simulink model "PerceptionAndGuidance"  (R2026b)
settings: Solver=ode3  StopTime=TFinal
PreLoadFcn:
  | InitVars;
libraries: raspberrypiutilitieslib x2, raspberrypiCommlib x2, simulink x1
settings Model: Creator=The MathWorks, Inc.  LastModifiedBy=rbhan
settings SolverCC: AutoInsertRateTranBlk=on  PositivePriorityOrder=on
settings OptimizationCC: DifferentSizesBufferReuse=on  EfficientTunableParamExpr=on  EnhancedBackFolding=on  MaxStackSize=200000  OptimizationCustomize=off  OptimizeBlockOrder=speed  PassReuseOutputArgsAs=Individual arguments  RemoveInternalMemoryZeroInit=on  RemoveRootLevelIOMemoryZeroInit=on
settings DebuggingCC: ParameterPrecisionLossMsg=none  ParameterTunabilityLossMsg=error
settings HardwareCC: ProdHWDeviceType=ARM Compatible->ARM Cortex-A (32-bit)  ProdLargestAtomicFloat=Double  ProdLargestAtomicInteger=Long  ProdLongLongMode=on
settings ModelReferenceCC: PropagateVarSize=During execution
settings RTWCC: BuildConfiguration=Faster Runs  Description=Embedded Coder  SystemTargetFile=ert.tlc  TemplateMakefile=ert_default_tmf
settings CodeAppCC: ForceParamTrailComments=on  IgnoreCustomStorageClasses=off  InsertBlockDesc=on  OperatorAnnotations=on  SFDataObjDesc=on  SimulinkDataObjDesc=on
settings ERTTargetCC: CodeReplacementLibrary=ARM Cortex-A CMSIS  ExtModeIntrfLevel=Level2 - Open  ExtModeMexFile=ext_xcp  ExtModeStaticAlloc=on  SupportVariableSizeSignals=on

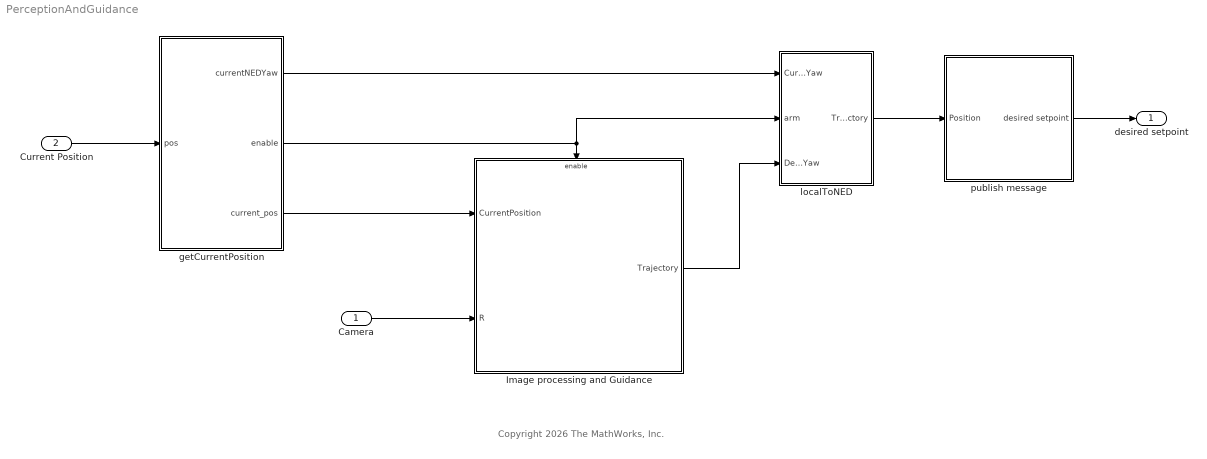
== system PerceptionAndGuidance ==
  note: Copyright 2026 The MathWorks, Inc.
  Camera : Inport  OutDataTypeStr=uint8  PortDimensions=[120 160 3]
  Current Position : Inport  Port=2  OutDataTypeStr=double  PortDimensions=4
  Image processing and Guidance : Subsystem
  getCurrentPosition : Subsystem  Variant=on
  localToNED : Subsystem
  publish message : Subsystem  Variant=on
  desired setpoint : Outport  OutDataTypeStr=Bus: desiredTargetSetpoints
  wires:
  localToNED/1(Trajectory) -> publish message/1(Position)
  getCurrentPosition/1(currentNEDYaw) -> localToNED/1(CurrentNEDYaw)
  Image processing and Guidance/1(Trajectory) -> localToNED/3(DesiredPosAndYaw)
  getCurrentPosition/2(enable) -> Image processing and Guidance/Enable, localToNED/2(arm)
  Camera/1 -> Image processing and Guidance/2(R)
  Current Position/1 -> getCurrentPosition/1(pos)
  getCurrentPosition/3(current_pos) -> Image processing and Guidance/1(CurrentPosition)
  publish message/1(desired setpoint) -> desired setpoint/1

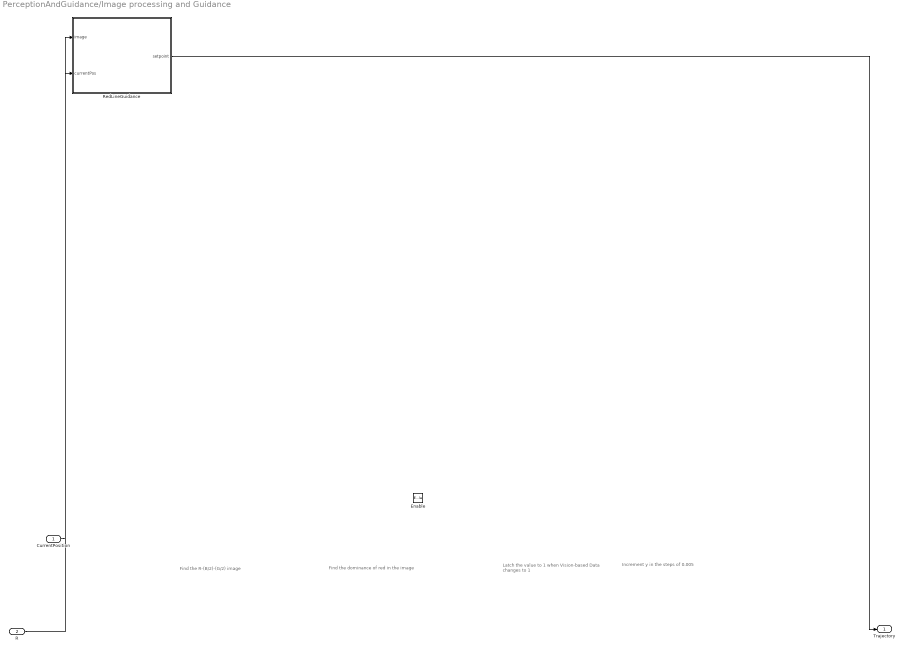
== system PerceptionAndGuidance/Image processing and Guidance ==
  note: Find the dominance of red in the image
  note: Increment y in the steps of 0.005
  note: Find the R-(B/2)-(G/2) image
  note: Latch the value to 1 when
      | Vision-based Data changes to 1
  CurrentPosition : Inport  OutDataTypeStr=double  PortDimensions=4
  R : Inport  Port=2  OutDataTypeStr=uint8  PortDimensions=[120 160 3]
  Enable : EnablePort
  RedLineGuidance : MATLAB Function  TreatAsAtomicUnit=on
  Trajectory : Outport
  wires:
  R/1 -> RedLineGuidance/1(image)
  CurrentPosition/1 -> RedLineGuidance/2(currentPos)
  RedLineGuidance/1(setpoint) -> Trajectory/1

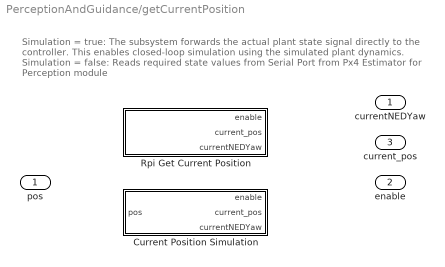
== system PerceptionAndGuidance/getCurrentPosition ==
  note: Simulation = true:
      | The subsystem forwards the actual plant state signal directly to the controller. This enables closed-loop simulation using the simulated plant dynamics.
      |
      | Simulation = false:
      | Reads required state values from Serial Port from Px4 Estimator for Perception module
  pos : Inport  PortDimensions=[1 4]
  Current Position Simulation : Subsystem  VariantControl=Simulation == true
  Rpi Get Current Position : Subsystem  VariantControl=Simulation == false
  currentNEDYaw : Outport
  enable : Outport  Port=2
  current_pos : Outport  Port=3

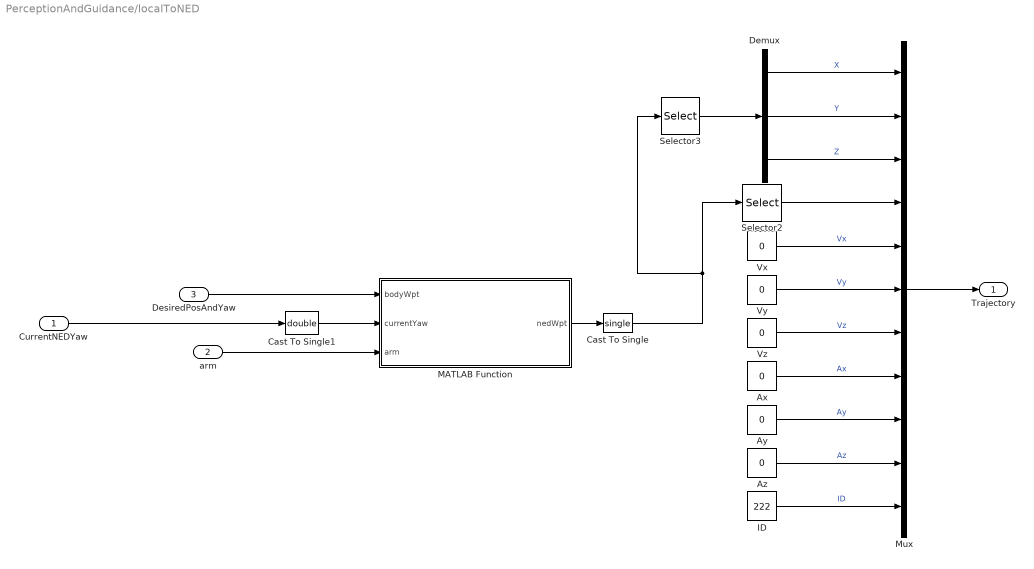
== system PerceptionAndGuidance/localToNED ==
  CurrentNEDYaw : Inport
  arm : Inport  Port=2
  DesiredPosAndYaw : Inport  Port=3
  Ax : Constant  Value=0  OutDataTypeStr=single  SampleTime=-1
  Ay : Constant  Value=0  OutDataTypeStr=single  SampleTime=-1
  Az : Constant  Value=0  OutDataTypeStr=single  SampleTime=-1
  Cast To Single : DataTypeConversion  OutDataTypeStr=single  SaturateOnIntegerOverflow=off  RndMeth=Floor
  Cast To Single1 : DataTypeConversion  OutDataTypeStr=double  SaturateOnIntegerOverflow=off  RndMeth=Floor
  Demux : Demux  Outputs=3
  ID : Constant  Value=222  OutDataTypeStr=single  SampleTime=-1
  MATLAB Function : MATLAB Function  TreatAsAtomicUnit=on
  Mux : Mux  Inputs=11
  Selector2 : Selector  InputPortWidth=4  IndexOptions=Index vector (dialog)  Indices=4  OutputSizes=1
  Selector3 : Selector  InputPortWidth=4  IndexOptions=Index vector (dialog)  Indices=[1:3]  OutputSizes=1
  Vx : Constant  Value=0  OutDataTypeStr=single  SampleTime=-1
  Vy : Constant  Value=0  OutDataTypeStr=single  SampleTime=-1
  Vz : Constant  Value=0  OutDataTypeStr=single  SampleTime=-1
  Trajectory : Outport
  wires:
  Selector3/1 -> Demux/1
  Mux/1 -> Trajectory/1
  Demux/2 -> Mux/2  "Y"
  Demux/3 -> Mux/3  "Z"
  Selector2/1 -> Mux/4
  Cast To Single/1 -> Selector3/1, Selector2/1
  ID/1 -> Mux/11  "ID"
  Demux/1 -> Mux/1  "X"
  Vx/1 -> Mux/5  "Vx"
  Vy/1 -> Mux/6  "Vy"
  Az/1 -> Mux/10  "Az"
  Vz/1 -> Mux/7  "Vz"
  Ay/1 -> Mux/9  "Ay"
  MATLAB Function/1(nedWpt) -> Cast To Single/1
  Ax/1 -> Mux/8  "Ax"
  DesiredPosAndYaw/1 -> MATLAB Function/1(bodyWpt)
  CurrentNEDYaw/1 -> Cast To Single1/1
  Cast To Single1/1 -> MATLAB Function/2(currentYaw)
  arm/1 -> MATLAB Function/3(arm)

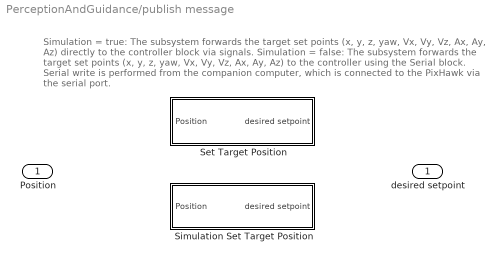
== system PerceptionAndGuidance/publish message ==
  note: Simulation = true:
      | The subsystem forwards the target set points (x, y, z, yaw, Vx, Vy, Vz, Ax, Ay, Az) directly to the controller block via signals.
      |
      | Simulation = false:
      | The subsystem forwards the target set points (x, y, z, yaw, Vx, Vy, Vz, Ax, Ay, Az) to the controller using the Serial block. Serial write is performed from the companion computer, which is connected to the PixHawk via the serial port.
  Position : Inport
  Set Target Position : Subsystem  VariantControl=Simulation == false
  Simulation Set Target Position : Subsystem  VariantControl=Simulation == true
  desired setpoint : Outport

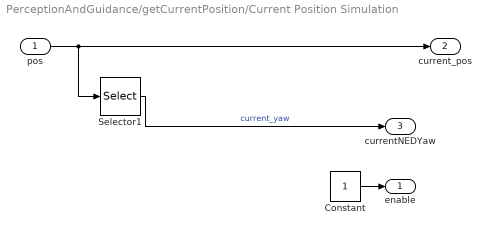
== system PerceptionAndGuidance/getCurrentPosition/Current Position Simulation ==
  pos : Inport
  Constant : Constant  SampleTime=-1
  Selector1 : Selector  InputPortWidth=4  IndexOptions=Index vector (dialog)  Indices=4  OutputSizes=1
  enable : Outport
  current_pos : Outport  Port=2
  currentNEDYaw : Outport  Port=3
  wires:
  pos/1 -> current_pos/1, Selector1/1
  Constant/1 -> enable/1
  Selector1/1 -> currentNEDYaw/1  "current_yaw"

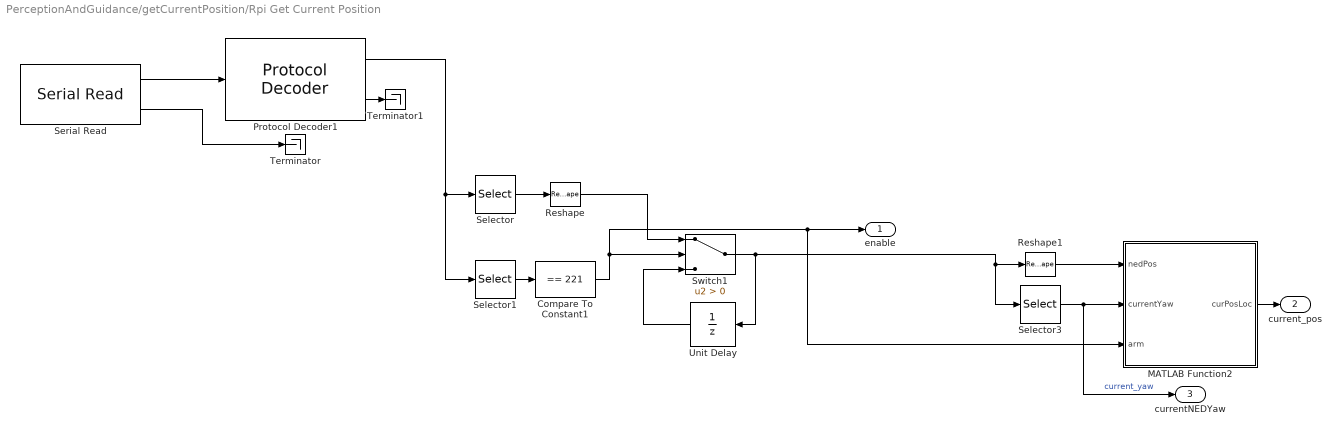
== system PerceptionAndGuidance/getCurrentPosition/Rpi Get Current Position ==
  Compare To Constant1 : simulink/Logic and Bit Operations/Compare To Constant  relop===  const=221  OutDataTypeStr=boolean
  MATLAB Function2 : MATLAB Function  TreatAsAtomicUnit=on
  Protocol Decoder1 : raspberrypiutilitieslib/Protocol Decoder  IsParseCSV=off  Header=[123]  FieldTable={ 'Field1', '5', 'single', 'Little endian' }  IsVariableSizeLastField=off  MaxVariableSizeFieldLength=[]  IsChecksumRequired=off  ChecksumAlgorithm=XOR of bytes  ChecksumSize=[]  TerminatorOption=<none>  CustomTerminatorVal=[]  IsInputLengthAvailable=off
  Reshape : Reshape
  Reshape1 : Reshape  OutputDimensionality=Customize  OutputDimensions=[4,1]
  Selector : Selector  InputPortWidth=5  IndexOptions=Index vector (dialog)  Indices=[1:4]  OutputSizes=1
  Selector1 : Selector  InputPortWidth=5  IndexOptions=Index vector (dialog)  Indices=[5]  OutputSizes=1
  Selector3 : Selector  InputPortWidth=4  IndexOptions=Index vector (dialog)  Indices=4  OutputSizes=1
  Serial Read : raspberrypiCommlib/Serial Read  board=Pi Zero W  SCIModule_=/dev/ttyACM0  Baudrate_=115200  Parity=None  StopBits_=1  HardwareFlowControl=None  ByteOrder=LittleEndian  DataLength=21  DataType=uint8  OutputStatus=on  SampleTime=0.1  blockPlatform=RaspberryPi
  Switch1 : Switch  Criteria=u2 > Threshold  SaturateOnIntegerOverflow=off  InputSameDT=off
  Terminator : Terminator
  Terminator1 : Terminator
  Unit Delay : UnitDelay  InitialCondition=[0 0 0 0]'  SampleTime=-1
  enable : Outport
  current_pos : Outport  Port=2
  currentNEDYaw : Outport  Port=3
  wires:
  Unit Delay/1 -> Switch1/3
  Serial Read/1 -> Protocol Decoder1/1
  Serial Read/2 -> Terminator/1
  Protocol Decoder1/1 -> Selector1/1, Selector/1
  Selector1/1 -> Compare To Constant1/1
  Selector/1 -> Reshape/1
  Reshape/1 -> Switch1/1
  Protocol Decoder1/2 -> Terminator1/1
  Selector3/1 -> currentNEDYaw/1, MATLAB Function2/2(currentYaw)  "current_yaw"
  Compare To Constant1/1 -> MATLAB Function2/3(arm), enable/1, Switch1/2
  Switch1/1 -> Unit Delay/1, Selector3/1, Reshape1/1
  Reshape1/1 -> MATLAB Function2/1(nedPos)
  MATLAB Function2/1(curPosLoc) -> current_pos/1

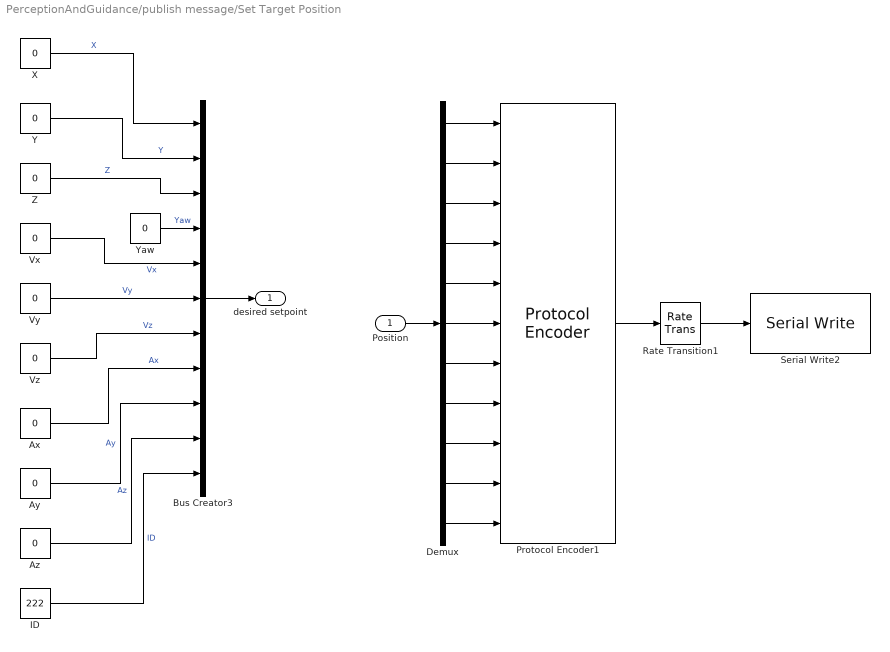
== system PerceptionAndGuidance/publish message/Set Target Position ==
  Position : Inport
  Ax : Constant  Value=0  SampleTime=-1
  Ay : Constant  Value=0  SampleTime=-1
  Az : Constant  Value=0  SampleTime=-1
  Bus Creator3 : BusCreator  Inputs=11  OutDataTypeStr=Bus: desiredTargetSetpoints
  Demux : Demux  Outputs=11
  ID : Constant  Value=222  SampleTime=-1
  Protocol Encoder1 : raspberrypiutilitieslib/Protocol Encoder  Header=[134]  FieldTable={ 'Field1', '1', 'single', 'Little endian'; 'Field2', '1', 'single', 'Little endian'; 'Field3', '1', 'single', 'Little endian'; 'Field4', '1', 'single', 'Little endian'; 'Field5', '1', 'single', 'Little endian'; 'Field6', '1', 'single', 'Little endian'; 'Field7', '1', 'single', 'Little endian'; 'Field8', '1', 'single', 'Little endian'; 'Field9', '1', 'single', 'Little endian'; 'Field10', '1', 'single', 'Little endian'; 'Field11', '1', 'single', 'Little endian' }  IsChecksumRequired=off  ChecksumAlgorithm=XOR of bytes  ChecksumSize=[]  TerminatorOption=<none>  CustomTerminatorVal=[]
  Rate Transition1 : RateTransition  OutPortSampleTime=1/10
  Serial Write2 : raspberrypiCommlib/Serial Write  board=Pi Zero W  SCIModule_=/dev/ttyACM0  Baudrate_=115200  Parity=None  StopBits_=1  HardwareFlowControl=None  ByteOrder=LittleEndian  OutputStatus=off  blockPlatform=RaspberryPi
  Vx : Constant  Value=0  SampleTime=-1
  Vy : Constant  Value=0  SampleTime=-1
  Vz : Constant  Value=0  SampleTime=-1
  X : Constant  Value=0  SampleTime=-1
  Y : Constant  Value=0  SampleTime=-1
  Yaw : Constant  Value=0  SampleTime=-1
  Z : Constant  Value=0  SampleTime=-1
  desired setpoint : Outport  OutDataTypeStr=Bus: desiredTargetSetpoints
  wires:
  Ax/1 -> Bus Creator3/8  "Ax"
  X/1 -> Bus Creator3/1  "X"
  Y/1 -> Bus Creator3/2  "Y"
  Z/1 -> Bus Creator3/3  "Z"
  Ay/1 -> Bus Creator3/9  "Ay"
  Vx/1 -> Bus Creator3/5  "Vx"
  Vy/1 -> Bus Creator3/6  "Vy"
  Vz/1 -> Bus Creator3/7  "Vz"
  Az/1 -> Bus Creator3/10  "Az"
  ID/1 -> Bus Creator3/11  "ID"
  Bus Creator3/1 -> desired setpoint/1
  Rate Transition1/1 -> Serial Write2/1
  Protocol Encoder1/1 -> Rate Transition1/1
  Demux/1 -> Protocol Encoder1/1
  Demux/2 -> Protocol Encoder1/2
  Demux/3 -> Protocol Encoder1/3
  Demux/4 -> Protocol Encoder1/4
  Demux/5 -> Protocol Encoder1/5
  Demux/6 -> Protocol Encoder1/6
  Demux/7 -> Protocol Encoder1/7
  Demux/8 -> Protocol Encoder1/8
  Demux/9 -> Protocol Encoder1/9
  Demux/10 -> Protocol Encoder1/10
  Demux/11 -> Protocol Encoder1/11
  Position/1 -> Demux/1
  Yaw/1 -> Bus Creator3/4  "Yaw"

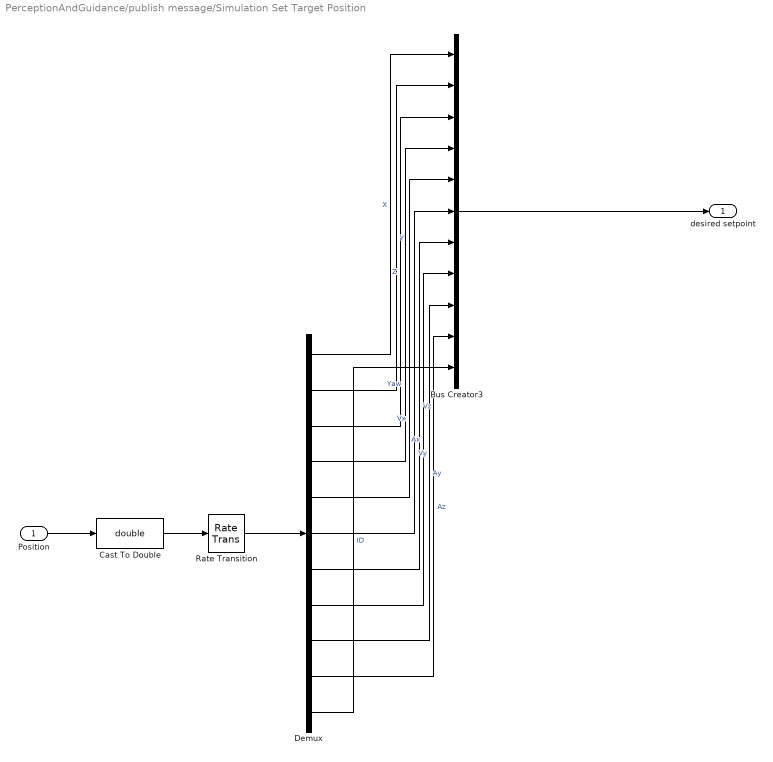
== system PerceptionAndGuidance/publish message/Simulation Set Target Position ==
  Position : Inport
  Bus Creator3 : BusCreator  Inputs=11  OutDataTypeStr=Bus: desiredTargetSetpoints
  Cast To Double : DataTypeConversion  OutDataTypeStr=double  SaturateOnIntegerOverflow=off  RndMeth=Floor
  Demux : Demux  Outputs=11
  Rate Transition : RateTransition  OutPortSampleTime=0.2
  desired setpoint : Outport  OutDataTypeStr=Bus: desiredTargetSetpoints
  wires:
  Demux/1 -> Bus Creator3/1  "X"
  Demux/2 -> Bus Creator3/2  "Y"
  Demux/3 -> Bus Creator3/3  "Z"
  Demux/4 -> Bus Creator3/4  "Yaw"
  Demux/5 -> Bus Creator3/5  "Vx"
  Demux/6 -> Bus Creator3/6  "Vy"
  Demux/7 -> Bus Creator3/7  "Vz"
  Demux/8 -> Bus Creator3/8  "Ax"
  Demux/9 -> Bus Creator3/9  "Ay"
  Demux/10 -> Bus Creator3/10  "Az"
  Demux/11 -> Bus Creator3/11  "ID"
  Position/1 -> Cast To Double/1
  Rate Transition/1 -> Demux/1
  Cast To Double/1 -> Rate Transition/1
  Bus Creator3/1 -> desired setpoint/1

== matlab function PerceptionAndGuidance/getCurrentPosition/Rpi Get Current Position/MATLAB Function2 ==
  data: nedPos input; curPosLoc output; currentYaw input; arm input
function curPosLoc = ned2body_waypoint(nedPos, currentYaw, arm)
% nedPos: 1x4 [x_ned, y_ned, z, yaw_ned]
% currentYaw: scalar (current yaw from PX4, in radians)
% arm: boolean (true if vehicle is armed)
% Output: 1x4 [x_body, y_body, z, yaw_body]

persistent yaw0 isLatched

if isempty(yaw0)
    yaw0 = single(0);
end
if isempty(isLatched)
    isLatched = false;
end

x_n = nedPos(1);
y_n = nedPos(2);
z_n = nedPos(3);
yaw_n = nedPos(4);

if arm && ~isLatched
    yaw0 = currentYaw;    % latch yaw when arming occurs
    isLatched = true;
elseif ~arm
    isLatched = false;    % reset latch if disarmed
end

if isLatched
    % Transform to body frame relative to yaw0
    x_b =  x_n * cos(yaw0) + y_n * sin(yaw0);
    y_b = -x_n * sin(yaw0) + y_n * cos(yaw0);
    yaw_b = wrapToPi(yaw_n - yaw0);
    curPosLoc = [x_b; y_b; z_n; yaw_b];
else
    % Not armed: just forward readings (no transform)
    curPosLoc = [x_n; y_n; z_n; yaw_n];
end
end

== matlab function PerceptionAndGuidance/localToNED/MATLAB Function ==
  data: bodyWpt input; nedWpt output; currentYaw input; arm input
function nedWpt = body2ned_waypoint(bodyWpt, currentYaw, arm)
%#codegen
nedWpt = double(reshape(bodyWpt, 4, 1));
end

== matlab function PerceptionAndGuidance/Image processing and Guidance/RedLineGuidance ==
  data: image input uint8 size=[120 160 3]; setpoint output double size=4; currentPos input double size=4
function setpoint = RedLineGuidance(image, currentPos)
%#codegen
% REDLINEGUIDANCE Robust closed-loop perception and guidance for MATLAB Minidrone Red Line Follower
%
% Fully autonomous guidance system designed to follow arbitrary red line tracks regardless of
% geometry: normal corners (90 deg), sharp acute corners (45-60 deg / hairpins), obtuse turns,
% smooth curves, line gaps, and distractors, with precision alignment and landing on the destination circle.
%
% Inputs:
%   image:      120x160x3 uint8 downward camera frame
%   currentPos: [X; Y; Z; yaw] drone state in NED frame
%
% Output:
%   setpoint:   [X_cmd; Y_cmd; Z_cmd; yaw_cmd] in NED frame

persistent state x_cmd y_cmd z_cmd yaw_cmd is_init
persistent last_valid_yaw loss_timer takeoff_timer align_timer landed_timer
persistent x0 y0 yaw0 circle_x circle_y
persistent corner_x corner_y corner_turn_dir turn_start_yaw
persistent circle_confirm_timer corner_cooldown incoming_yaw
persistent turn_score

% State definitions:
% 0: TAKEOFF / CLIMB
% 1: TRACK (Lookahead pursuit for straight lines and gentle curves)
% 2: APPROACH_CORNER (Straight-line deceleration into corner vertex, zero lateral drift, zero overshoot)
% 3: CORNER_TURN (In-place yaw rotation holding corner vertex, handles 45-160 deg turns)
% 4: GAP_RECOVER (Crawl along last heading if line temporarily lost)
% 5: ALIGN_CIRCLE (Precision 2D centering over destination circle)
% 6: LAND (Active descent with closed-loop centering)
% 7: LANDED (Touchdown hold)

dt = 0.20;          % Camera frame period (5 Hz)
CRUISE_ALT = -0.80; % Cruise altitude (0.8m above ground)

if isempty(is_init)
    state = 0;
    x0 = currentPos(1);
    y0 = currentPos(2);
    yaw0 = currentPos(4);
    x_cmd = x0;
    y_cmd = y0;
    z_cmd = CRUISE_ALT;
    yaw_cmd = yaw0;
    last_valid_yaw = yaw0;
    incoming_yaw = yaw0;
    circle_x = x0;
    circle_y = y0;
    corner_x = x0;
    corner_y = y0;
    corner_turn_dir = 1;
    turn_start_yaw = yaw0;
    loss_timer = 0;
    takeoff_timer = 0;
    align_timer = 0;
    landed_timer = 0;
    circle_confirm_timer = 0;
    corner_cooldown = 0;
    turn_score = 0;
    is_init = true;
end

% Decrement corner cooldown timer
if corner_cooldown > 0
    corner_cooldown = max(0, corner_cooldown - dt);
end

% Extract RGB color channels
R = double(image(:,:,1));
G = double(image(:,:,2));
B = double(image(:,:,3));

% 1. Robust Red Pixel Segmentation
% Rejects gravel floor (grey/green), yellow distractors (R~G), blue distractors, and shadows
is_red = (R > 75) & ...
         (R - G > 25) & ...
         (R - B > 25) & ...
         (R ./ max(G + B, 1) > 0.65);

nRed = sum(is_red(:));

% Altitude-adaptive metric scaling (meters per pixel)
curr_h = max(-currentPos(3), 0.15);
scale = 0.00432 * (curr_h / 0.80);

% 2. Image Feature Extraction
% Camera frame geometry:
% Row 1 = Forward (+X body), Row 120 = Rear (-X body), Row 60 = Nadir (drone center)
% Col 1 = Left (-Y body), Col 160 = Right (+Y body), Col 80 = Centerline

[rAll, cAll] = find(is_red);
if ~isempty(rAll)
    c_all = mean(cAll);
    r_all = mean(rAll);
    min_c = min(cAll);
    max_c = max(cAll);
    min_r = min(rAll);
    max_r = max(rAll);
    r_span = max_r - min_r;
    c_span = max_c - min_c;
else
    c_all = 80; r_all = 60;
    min_c = 80; max_c = 80; min_r = 60; max_r = 60;
    r_span = 0; c_span = 0;
end

% Regional zoning:
% Mid zone: rows 39 to 68 (primary corridor anchor)
maskMid = is_red(39:68, :);
[rM, cM] = find(maskMid);
nMid = length(cM);
if ~isempty(cM)
    % Centerline corridor: reject distant old legs / acute angle wedge distractors
    cM_corridor = cM(abs(cM - 80) < 38);
    rM_corridor = rM(abs(cM - 80) < 38);
    if ~isempty(cM_corridor)
        c_mid = mean(cM_corridor);
        r_mid = mean(rM_corridor) + 38;
    else
        c_mid = mean(cM);
        r_mid = mean(rM) + 38;
    end
else
    c_mid = c_all;
    r_mid = 54;
end

% Forward zone: rows 10 to 38
maskFar = is_red(10:38, :);
[rF, cF] = find(maskFar);
nFar = length(cF);
if ~isempty(cF)
    cF_corridor = cF(abs(cF - c_mid) < 38);
    rF_corridor = rF(abs(cF - c_mid) < 38);
    if ~isempty(cF_corridor)
        c_far = mean(cF_corridor);
        r_far = mean(rF_corridor) + 9;
    else
        c_far = mean(cF);
        r_far = mean(rF) + 9;
    end
    c_span_far = max(cF) - min(cF);
    min_c_far = min(cF);
    max_c_far = max(cF);
else
    c_far = 80;
    r_far = 24;
    c_span_far = 0;
    min_c_far = 80;
    max_c_far = 80;
end

% Near / Base zone: rows 60 to 95 (directly beneath drone)
maskNear = is_red(60:95, :);
[rN, cN] = find(maskNear);
nNear = length(cN);
if ~isempty(cN)
    cN_corridor = cN(abs(cN - c_mid) < 38);
    rN_corridor = rN(abs(cN - c_mid) < 38);
    if ~isempty(cN_corridor)
        c_near = mean(cN_corridor);
        r_near = mean(rN_corridor) + 59;
    else
        c_near = mean(cN);
        r_near = mean(rN) + 59;
    end
else
    c_near = c_all;
    r_near = r_all;
end

% Side branch detection: line extends towards side image boundaries
isSideBranch = (max_c >= 152) || (min_c <= 8);

% Vector from mid to forward path (lookahead vector, completely immune to rear/incoming track):
dr_fwd = max(r_mid - r_far, 1);
dc_fwd = c_far - c_mid;
psi_fwd = atan2(dc_fwd, dr_fwd);

% Vector from near base to forward path:
dr_line = max(r_near - r_far, 1);
dc_line = c_far - c_near;
psi_line = atan2(dc_line, dr_line);

% Lateral offset of track ahead of drone (using mid zone row ~54):
lat_err = (c_mid - 80) * scale; % meters

% 3. Robust Landing Circle Discrimination
% Dedicated circle inspection zone (rows 10 to 80)
maskCircle = is_red(10:80, :);
[rC, cC] = find(maskCircle);
nCircle = length(cC);
if ~isempty(cC)
    r_span_c = max(rC) - min(rC);
    c_span_c = max(cC) - min(cC);
    min_c_c = min(cC);
    max_c_c = max(cC);
    fill_factor_c = nCircle / max(r_span_c * c_span_c, 1);
else
    r_span_c = 0; c_span_c = 0;
    min_c_c = 80; max_c_c = 80;
    fill_factor_c = 0;
end

is_circle_candidate = (nCircle >= 500) && (nCircle <= 2400) && ...
                      (r_span_c >= 25) && (r_span_c <= 62) && ...
                      (c_span_c >= 35) && (c_span_c <= 58) && ...
                      (abs(r_span_c - c_span_c) <= 18) && ...
                      (fill_factor_c >= 0.52) && ...
                      (min_c_c > 18) && (max_c_c < 142) && ...
                      (corner_cooldown <= 0) && ...
                      (state == 1 || state == 2 || state == 4);

if is_circle_candidate
    circle_confirm_timer = circle_confirm_timer + dt;
else
    circle_confirm_timer = max(0, circle_confirm_timer - 2 * dt);
end

% Circle confirmed only after persistent detection across multiple frames
isCircle = (circle_confirm_timer >= 0.20);

% 4. Corner & Sharp Turn Detection (Early Lookahead Detection)
% Detects 90-degree corners, acute angles, and obtuse turns BEFORE reaching the vertex:
isCornerAhead = (corner_cooldown <= 0) && ~is_circle_candidate && ...
                (((nFar < 35) && (nMid > 45) && (isSideBranch || c_span > 75)) || ...
                 ((c_span_far > 40) && (nFar > 45) && (min_c_far < 20 || max_c_far > 140)) || ...
                 ((abs(psi_line) > deg2rad(28)) && (nFar > 40) && (isSideBranch || c_span > 50)));

% Is the drone currently AT the corner vertex?
% The forward line has ended directly at nadir (rows 10-38 empty) while the corner is directly underneath
isAtCorner = (corner_cooldown <= 0) && ~is_circle_candidate && (nFar < 20) && (nNear > 50) && (isSideBranch || c_span > 75);

% 5. Finite State Machine Execution
if state == 0 % TAKEOFF / CLIMB
    z_cmd = CRUISE_ALT;
    x_cmd = x0;
    y_cmd = y0;
    yaw_cmd = yaw0;
    last_valid_yaw = yaw0;
    incoming_yaw = yaw0;
    
    takeoff_timer = takeoff_timer + dt;
    if (currentPos(3) <= (CRUISE_ALT + 0.15)) && (takeoff_timer >= 2.0)
        state = 1; % Enter regular track following
        loss_timer = 0;
    end

elseif state == 1 % LINE TRACKING (Straight lines & gentle curves)
    z_cmd = CRUISE_ALT;
    
    if isCircle
        state = 5; % Enter ALIGN_CIRCLE
        align_timer = 0;
        circle_x = currentPos(1);
        circle_y = currentPos(2);
    elseif isCornerAhead
        state = 2; % Enter APPROACH_CORNER (smooth straight-line deceleration into vertex)
        incoming_yaw = yaw_cmd; % Record the incoming straight heading
        turn_score = 0; % Reset turn direction evidence
    elseif nRed < 35
        loss_timer = loss_timer + dt;
        if loss_timer > 0.4
            state = 4; % Enter GAP_RECOVER
        end
    else
        loss_timer = 0;
        
        v_cruise = 0.25; % Cruise speed (m/s)
        
        % Lookahead heading error (forward-looking FOV, immune to rear vertices):
        psi_err = psi_fwd;
        
        % Adaptive speed based on alignment and lateral centering
        v_fwd = v_cruise * max(0.25, cos(psi_err))^2 * max(0.40, 1.0 - abs(lat_err) / 0.15);
        
        % Yaw rate command
        yaw_rate = 1.4 * psi_err;
        yaw_cmd = yaw_cmd + yaw_rate * dt;
        last_valid_yaw = yaw_cmd;
        
        % Body frame displacement setpoint
        dx_b = v_fwd * dt;
        dy_b = 0.65 * lat_err * dt + 0.25 * (c_far - 80) * scale * dt;
        
        % Convert body displacements to NED world frame
        cy = cos(yaw_cmd);
        sy = sin(yaw_cmd);
        x_cmd = x_cmd + (dx_b * cy - dy_b * sy);
        y_cmd = y_cmd + (dx_b * sy + dy_b * cy);
    end

elseif state == 2 % APPROACH_CORNER (Straight-line deceleration into corner vertex)
    z_cmd = CRUISE_ALT;
    
    % Accumulate branch evidence during the approach:
    % Pixels with c > 96 are on the RIGHT of incoming track centerline
    % Pixels with c < 64 are on the LEFT of incoming track centerline
    % (Incoming track is centered at col 80, width ~23 px, spanning cols 68:92, so it never reaches these thresholds!)
    nRight = sum(cAll > 96);
    nLeft  = sum(cAll < 64);
    turn_score = turn_score + (double(nRight) - double(nLeft));
    
    if isCircle
        state = 5; % Enter ALIGN_CIRCLE
        align_timer = 0;
        circle_x = currentPos(1);
        circle_y = currentPos(2);
    elseif isAtCorner || (nFar < 16)
        % Arrived at the corner vertex! Lock position and begin in-place rotation
        state = 3; % Enter CORNER_TURN
        corner_x = currentPos(1);
        corner_y = currentPos(2);
        turn_start_yaw = yaw_cmd;
        
        % Final branch check at vertex (evaluates both sides across full frame)
        nBranchRight = sum(cAll > 96);
        nBranchLeft  = sum(cAll < 64);
        
        if (turn_score > 30) || (nBranchRight > (nBranchLeft + 15))
            corner_turn_dir = 1;  % Turn Right (CW)
        elseif (turn_score < -30) || (nBranchLeft > (nBranchRight + 15))
            corner_turn_dir = -1; % Turn Left (CCW)
        elseif nBranchRight >= nBranchLeft
            corner_turn_dir = 1;
        else
            corner_turn_dir = -1;
        end
    else
        % CRITICAL FIX: Maintain straight heading along incoming line while decelerating!
        % DO NOT steer sideways into the branch before reaching the vertex!
        v_crawl = 0.08; % Slow glide into the corner (zero momentum overshoot)
        
        % Hold the incoming straight-line yaw heading
        yaw_cmd = incoming_yaw;
        last_valid_yaw = incoming_yaw;
        
        % Stay centered laterally over the incoming track centerline ONLY!
        % Side branch pixels (c > 96 or c < 64) MUST NOT corrupt lateral centering!
        cN_incoming = cN(cN >= 64 & cN <= 96);
        if ~isempty(cN_incoming)
            c_near_incoming = mean(cN_incoming);
        else
            c_near_incoming = 80;
        end
        lat_err_incoming = (c_near_incoming - 80) * scale;
        
        dx_b = v_crawl * dt;
        dy_b = 0.35 * lat_err_incoming * dt;
        
        cy = cos(yaw_cmd);
        sy = sin(yaw_cmd);
        x_cmd = x_cmd + (dx_b * cy - dy_b * sy);
        y_cmd = y_cmd + (dx_b * sy + dy_b * cy);
    end

elseif state == 3 % CORNER_TURN (In-place yaw rotation holding corner vertex)
    % 1. Firmly lock position setpoint at the corner vertex: prevents overshoot & backward drift
    x_cmd = corner_x;
    y_cmd = corner_y;
    z_cmd = CRUISE_ALT;
    
    % Unwrapped yaw turned so far
    yaw_turned = abs(atan2(sin(yaw_cmd - turn_start_yaw), cos(yaw_cmd - turn_start_yaw)));
    
    % 2. Adaptive dual-speed yaw rate:
    % Coarse slew: 0.80 rad/s (~46 deg/s) while turning towards branch
    % Fine capture: 0.28 rad/s (~16 deg/s) once branch appears in forward view (prevents overshooting the line!)
    if (yaw_turned >= deg2rad(25)) && (nFar > 25)
        yaw_rate = 0.28;
    else
        yaw_rate = 0.80;
    end
    
    yaw_cmd = yaw_cmd + corner_turn_dir * yaw_rate * dt;
    last_valid_yaw = yaw_cmd;
    
    % Recalculate yaw_turned after update
    yaw_turned = abs(atan2(sin(yaw_cmd - turn_start_yaw), cos(yaw_cmd - turn_start_yaw)));
    
    % 3. Check for alignment with the new branch:
    % Minimum 30 deg rotation prevents false early lock on incoming leg
    isAlignedWithNewBranch = (yaw_turned >= deg2rad(30)) && ...
                            (nFar > 35) && (nMid > 40) && ...
                            (abs(c_far - 80) < 18) && ...
                            (abs(psi_fwd) < deg2rad(15));
    
    if isAlignedWithNewBranch
        state = 1; % Aligned with new branch! Resume forward line tracking
        x_cmd = currentPos(1); % Smooth re-anchor from actual position
        y_cmd = currentPos(2);
        yaw_cmd = yaw_cmd + 0.50 * psi_fwd; % Fine snap heading to line
        last_valid_yaw = yaw_cmd;
        corner_cooldown = 2.5; % Prevent re-triggering corner on the same vertex
        loss_timer = 0;
        turn_score = 0;
    end

elseif state == 4 % GAP RECOVERY (Crawl forward across track gap)
    loss_timer = loss_timer + dt;
    v_crawl = 0.08;
    cy = cos(last_valid_yaw);
    sy = sin(last_valid_yaw);
    x_cmd = x_cmd + v_crawl * dt * cy;
    y_cmd = y_cmd + v_crawl * dt * sy;
    z_cmd = CRUISE_ALT;
    yaw_cmd = last_valid_yaw;
    
    if isCircle
        state = 5; % Enter ALIGN_CIRCLE
        align_timer = 0;
        circle_x = currentPos(1);
        circle_y = currentPos(2);
    elseif nRed > 70
        state = 1; % Reacquired red track
        loss_timer = 0;
    elseif loss_timer > 12.0
        % Safety emergency touchdown if track lost completely for > 12 seconds (~1m crawl)
        state = 6;
        circle_x = currentPos(1);
        circle_y = currentPos(2);
    end

elseif state == 5 % ALIGN OVER CIRCLE (Precision 2D centering over landing disc)
    if nCircle > 300
        r_circ = mean(rC) + 9;
        c_circ = mean(cC);
        dx_b = (60 - r_circ) * scale;
        dy_b = (c_circ - 80) * scale;
    else
        dx_b = (60 - r_all) * scale;
        dy_b = (c_all - 80) * scale;
    end
    cy = cos(last_valid_yaw);
    sy = sin(last_valid_yaw);
    
    % Smooth proportional centering over disc
    circle_x = currentPos(1) + 0.40 * (dx_b * cy - dy_b * sy);
    circle_y = currentPos(2) + 0.40 * (dx_b * sy + dy_b * cy);
    x_cmd = circle_x;
    y_cmd = circle_y;
    z_cmd = CRUISE_ALT;
    yaw_cmd = last_valid_yaw;
    
    align_timer = align_timer + dt;
    isCentered = (abs(dx_b) < 0.05) && (abs(dy_b) < 0.05);
    if (align_timer >= 0.6 && isCentered) || (align_timer >= 1.6)
        state = 6; % Centered! Start descent
    end

elseif state == 6 % CONTROLLED LANDING DESCENT (Active centering while descending)
    if nCircle > 300
        r_circ = mean(rC) + 9;
        c_circ = mean(cC);
        dx_b = (60 - r_circ) * scale;
        dy_b = (c_circ - 80) * scale;
    else
        dx_b = (60 - r_all) * scale;
        dy_b = (c_all - 80) * scale;
    end
    cy = cos(last_valid_yaw);
    sy = sin(last_valid_yaw);
    
    if nRed > 120
        circle_x = currentPos(1) + 0.25 * (dx_b * cy - dy_b * sy);
        circle_y = currentPos(2) + 0.25 * (dx_b * sy + dy_b * cy);
    end
    x_cmd = circle_x;
    y_cmd = circle_y;
    yaw_cmd = last_valid_yaw;
    
    z_cmd = min(0.04, z_cmd + 0.22 * dt); % Smooth 0.22 m/s descent
    if currentPos(3) > -0.06
        state = 7; % Touchdown complete
    end

elseif state == 7 % LANDED
    x_cmd = circle_x;
    y_cmd = circle_y;
    z_cmd = 0.05; % Hold firmly on ground
    yaw_cmd = last_valid_yaw;
    
    % Settle timer on the ground
    if currentPos(3) > -0.06
        landed_timer = landed_timer + dt;
    end
    
    % Once firmly landed and settled for 2.0s, signal simulation completion!
    if landed_timer >= 2.0
        z_cmd = 99.0; % MISSION COMPLETE: Landed and settled on target circle!
    end
end

setpoint = [x_cmd; y_cmd; z_cmd; yaw_cmd];
end
